simulink model "fft_biplex_real_4x_delay_bram_test"  (Simulink 7.4)
settings: Solver=VariableStepDiscrete  StartTime=0.0  StopTime=256  RelTol=1e-3
libraries: xbsIndex_r4 x596, casper_library_misc x36, casper_library_delays x8, casper_library_ffts_twiddle x1, simulink x1
(part 2 of 6)

== system fft_biplex_real_4x_delay_bram_test/fft_biplex_real_4x/bi_real_unscr_4x/hilbert0 ==
  a : Inport  OutDataType=sfix(16)  OutScaling=2^0
  b : Inport  Port=2  OutDataType=sfix(16)  OutScaling=2^0
  AddSub : xbsIndex_r4/AddSub  mode=Addition  use_carryin=off  use_carryout=off  en=off  latency=add_latency  precision=Full  arith_type=Unsigned  n_bits=8  bin_pt=2  quantization=Truncate  overflow=Wrap  dbl_ovrd=off  use_behavioral_HDL=on  hw_selection=Fabric  pipelined=off  use_rpm=on  block_type=addsub
      settings: xl_area=[0, 0, 0, 0, 0, 0, 0]  block_version=9.1.01
  AddSub1 : xbsIndex_r4/AddSub  mode=Subtraction  use_carryin=off  use_carryout=off  en=off  latency=add_latency  precision=Full  arith_type=Unsigned  n_bits=8  bin_pt=2  quantization=Truncate  overflow=Wrap  dbl_ovrd=off  use_behavioral_HDL=on  hw_selection=Fabric  pipelined=off  use_rpm=on  block_type=addsub
      settings: xl_area=[0, 0, 0, 0, 0, 0, 0]  block_version=9.1.01
  AddSub2 : xbsIndex_r4/AddSub  mode=Subtraction  use_carryin=off  use_carryout=off  en=off  latency=add_latency  precision=Full  arith_type=Unsigned  n_bits=8  bin_pt=2  quantization=Truncate  overflow=Wrap  dbl_ovrd=off  use_behavioral_HDL=on  hw_selection=Fabric  pipelined=off  use_rpm=on  block_type=addsub
      settings: xl_area=[0, 0, 0, 0, 0, 0, 0]  block_version=9.1.01
  AddSub3 : xbsIndex_r4/AddSub  mode=Addition  use_carryin=off  use_carryout=off  en=off  latency=add_latency  precision=Full  arith_type=Unsigned  n_bits=8  bin_pt=2  quantization=Truncate  overflow=Wrap  dbl_ovrd=off  use_behavioral_HDL=on  hw_selection=Fabric  pipelined=off  use_rpm=on  block_type=addsub
      settings: xl_area=[0, 0, 0, 0, 0, 0, 0]  block_version=9.1.01
  Convert{,1..3} (4 alike) : xbsIndex_r4/Convert  arith_type="Signed  (2's comp)"  n_bits=BitWidth  bin_pt=BitWidth - 1  quantization="Round  (unbiased: Even Values)"  overflow=Wrap  latency=conv_latency  dbl_ovrd=off  pipeline=off  block_type=convert
      settings: xl_area=[0, 0, 0, 0, 0, 0, 0]
  Scale{,1..3} (4 alike) : xbsIndex_r4/Scale  scale_factor=-1  dbl_ovrd=off  block_type=scale
  c_to_ri : Subsystem  AncestorBlock=casper_library_misc/c_to_ri  mask(c_to_ri){n_bits=BitWidth, bin_pt=BitWidth-1}
      mask prompts: n_bits "Bit Width"; bin_pt "Binary Point"
      mask help:
      | Outputs real and imaginary components of a complex input.
      | Useful for simplifying interconnects.
      | See also: Real-Imag to Complex (ri_to_c)
      mask init:
      | annotation=sprintf('%d_%d r/i',n_bits,bin_pt);
      | set_param(gcb,'AttributesFormatString',annotation);
      settings: AttributesFormatString=18_17 r/i
      mask Help: eval('xlWeb(''http://casper.berkeley.edu/wiki/C_to_ri'')')
  c_to_ri1 : Subsystem  AncestorBlock=casper_library_misc/c_to_ri  mask(c_to_ri){n_bits=BitWidth, bin_pt=BitWidth-1}
      mask prompts: n_bits "Bit Width"; bin_pt "Binary Point"
      mask help:
      | Outputs real and imaginary components of a complex input.
      | Useful for simplifying interconnects.
      | See also: Real-Imag to Complex (ri_to_c)
      mask init:
      | annotation=sprintf('%d_%d r/i',n_bits,bin_pt);
      | set_param(gcb,'AttributesFormatString',annotation);
      settings: AttributesFormatString=18_17 r/i
      mask Help: eval('xlWeb(''http://casper.berkeley.edu/wiki/C_to_ri'')')
  ri_to_c : Subsystem  AncestorBlock=casper_library_misc/ri_to_c
      mask Type: ri_to_c
      mask Description:
      | Concatenates real and imaginary inputs into a complex output.
      | Useful for simplifying interconnects.
      | See also: Complex to Real-Imag (c_to_ri)
      mask Help: eval('xlWeb(''http://casper.berkeley.edu/wiki/Ri_to_c'')')
  ri_to_c1 : Subsystem  AncestorBlock=casper_library_misc/ri_to_c
      mask Type: ri_to_c
      mask Description:
      | Concatenates real and imaginary inputs into a complex output.
      | Useful for simplifying interconnects.
      | See also: Complex to Real-Imag (c_to_ri)
      mask Help: eval('xlWeb(''http://casper.berkeley.edu/wiki/Ri_to_c'')')
  even : Outport  OutDataType=sfix(16)  OutScaling=2^0
  odd : Outport  Port=2  OutDataType=sfix(16)  OutScaling=2^0
  wires:
  Convert3/1 -> ri_to_c1/1(re)
  Convert1/1 -> ri_to_c1/2(im)
  AddSub/1 -> Scale/1
  AddSub1/1 -> Scale1/1
  AddSub2/1 -> Scale2/1
  AddSub3/1 -> Scale3/1
  c_to_ri/1(re) -> AddSub1/2, AddSub/1
  c_to_ri/2(im) -> AddSub2/1, AddSub3/1
  c_to_ri1/1(re) -> AddSub1/1, AddSub/2
  c_to_ri1/2(im) -> AddSub2/2, AddSub3/2
  Convert/1 -> ri_to_c/1(re)
  Convert2/1 -> ri_to_c/2(im)
  a/1 -> c_to_ri/1(c)
  ri_to_c/1(c) -> even/1
  ri_to_c1/1(c) -> odd/1
  b/1 -> c_to_ri1/1(c)
  Scale/1 -> Convert/1
  Scale1/1 -> Convert1/1
  Scale2/1 -> Convert2/1
  Scale3/1 -> Convert3/1

== system fft_biplex_real_4x_delay_bram_test/fft_biplex_real_4x/bi_real_unscr_4x/hilbert1 ==
  a : Inport  OutDataType=sfix(16)  OutScaling=2^0
  b : Inport  Port=2  OutDataType=sfix(16)  OutScaling=2^0
  AddSub : xbsIndex_r4/AddSub  mode=Addition  use_carryin=off  use_carryout=off  en=off  latency=add_latency  precision=Full  arith_type=Unsigned  n_bits=8  bin_pt=2  quantization=Truncate  overflow=Wrap  dbl_ovrd=off  use_behavioral_HDL=on  hw_selection=Fabric  pipelined=off  use_rpm=on  block_type=addsub
      settings: xl_area=[0, 0, 0, 0, 0, 0, 0]  block_version=9.1.01
  AddSub1 : xbsIndex_r4/AddSub  mode=Subtraction  use_carryin=off  use_carryout=off  en=off  latency=add_latency  precision=Full  arith_type=Unsigned  n_bits=8  bin_pt=2  quantization=Truncate  overflow=Wrap  dbl_ovrd=off  use_behavioral_HDL=on  hw_selection=Fabric  pipelined=off  use_rpm=on  block_type=addsub
      settings: xl_area=[0, 0, 0, 0, 0, 0, 0]  block_version=9.1.01
  AddSub2 : xbsIndex_r4/AddSub  mode=Subtraction  use_carryin=off  use_carryout=off  en=off  latency=add_latency  precision=Full  arith_type=Unsigned  n_bits=8  bin_pt=2  quantization=Truncate  overflow=Wrap  dbl_ovrd=off  use_behavioral_HDL=on  hw_selection=Fabric  pipelined=off  use_rpm=on  block_type=addsub
      settings: xl_area=[0, 0, 0, 0, 0, 0, 0]  block_version=9.1.01
  AddSub3 : xbsIndex_r4/AddSub  mode=Addition  use_carryin=off  use_carryout=off  en=off  latency=add_latency  precision=Full  arith_type=Unsigned  n_bits=8  bin_pt=2  quantization=Truncate  overflow=Wrap  dbl_ovrd=off  use_behavioral_HDL=on  hw_selection=Fabric  pipelined=off  use_rpm=on  block_type=addsub
      settings: xl_area=[0, 0, 0, 0, 0, 0, 0]  block_version=9.1.01
  Convert{,1..3} (4 alike) : xbsIndex_r4/Convert  arith_type="Signed  (2's comp)"  n_bits=BitWidth  bin_pt=BitWidth - 1  quantization="Round  (unbiased: Even Values)"  overflow=Wrap  latency=conv_latency  dbl_ovrd=off  pipeline=off  block_type=convert
      settings: xl_area=[0, 0, 0, 0, 0, 0, 0]
  Scale{,1..3} (4 alike) : xbsIndex_r4/Scale  scale_factor=-1  dbl_ovrd=off  block_type=scale
  c_to_ri : Subsystem  AncestorBlock=casper_library_misc/c_to_ri  mask(c_to_ri){n_bits=BitWidth, bin_pt=BitWidth-1}
      mask prompts: n_bits "Bit Width"; bin_pt "Binary Point"
      mask help:
      | Outputs real and imaginary components of a complex input.
      | Useful for simplifying interconnects.
      | See also: Real-Imag to Complex (ri_to_c)
      mask init:
      | annotation=sprintf('%d_%d r/i',n_bits,bin_pt);
      | set_param(gcb,'AttributesFormatString',annotation);
      settings: AttributesFormatString=18_17 r/i
      mask Help: eval('xlWeb(''http://casper.berkeley.edu/wiki/C_to_ri'')')
  c_to_ri1 : Subsystem  AncestorBlock=casper_library_misc/c_to_ri  mask(c_to_ri){n_bits=BitWidth, bin_pt=BitWidth-1}
      mask prompts: n_bits "Bit Width"; bin_pt "Binary Point"
      mask help:
      | Outputs real and imaginary components of a complex input.
      | Useful for simplifying interconnects.
      | See also: Real-Imag to Complex (ri_to_c)
      mask init:
      | annotation=sprintf('%d_%d r/i',n_bits,bin_pt);
      | set_param(gcb,'AttributesFormatString',annotation);
      settings: AttributesFormatString=18_17 r/i
      mask Help: eval('xlWeb(''http://casper.berkeley.edu/wiki/C_to_ri'')')
  ri_to_c : Subsystem  AncestorBlock=casper_library_misc/ri_to_c
      mask Type: ri_to_c
      mask Description:
      | Concatenates real and imaginary inputs into a complex output.
      | Useful for simplifying interconnects.
      | See also: Complex to Real-Imag (c_to_ri)
      mask Help: eval('xlWeb(''http://casper.berkeley.edu/wiki/Ri_to_c'')')
  ri_to_c1 : Subsystem  AncestorBlock=casper_library_misc/ri_to_c
      mask Type: ri_to_c
      mask Description:
      | Concatenates real and imaginary inputs into a complex output.
      | Useful for simplifying interconnects.
      | See also: Complex to Real-Imag (c_to_ri)
      mask Help: eval('xlWeb(''http://casper.berkeley.edu/wiki/Ri_to_c'')')
  even : Outport  OutDataType=sfix(16)  OutScaling=2^0
  odd : Outport  Port=2  OutDataType=sfix(16)  OutScaling=2^0
  wires:
  Convert3/1 -> ri_to_c1/1(re)
  Convert1/1 -> ri_to_c1/2(im)
  AddSub/1 -> Scale/1
  AddSub1/1 -> Scale1/1
  AddSub2/1 -> Scale2/1
  AddSub3/1 -> Scale3/1
  c_to_ri/1(re) -> AddSub1/2, AddSub/1
  c_to_ri/2(im) -> AddSub2/1, AddSub3/1
  c_to_ri1/1(re) -> AddSub1/1, AddSub/2
  c_to_ri1/2(im) -> AddSub2/2, AddSub3/2
  Convert/1 -> ri_to_c/1(re)
  Convert2/1 -> ri_to_c/2(im)
  a/1 -> c_to_ri/1(c)
  ri_to_c/1(c) -> even/1
  ri_to_c1/1(c) -> odd/1
  b/1 -> c_to_ri1/1(c)
  Scale/1 -> Convert/1
  Scale1/1 -> Convert1/1
  Scale2/1 -> Convert2/1
  Scale3/1 -> Convert3/1

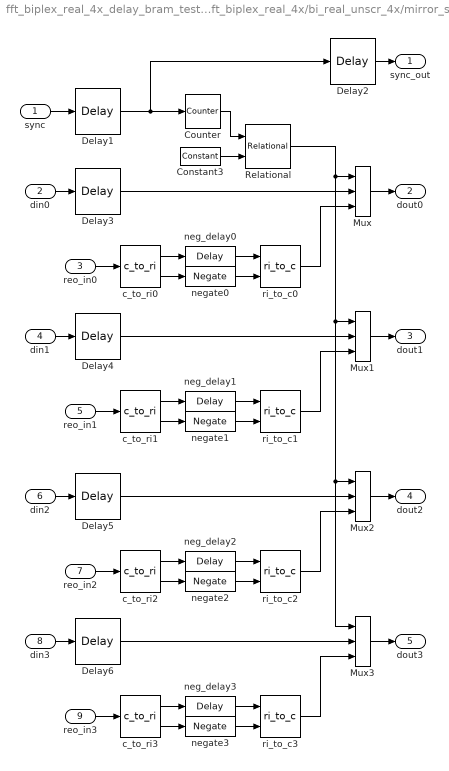
== system fft_biplex_real_4x_delay_bram_test/fft_biplex_real_4x/bi_real_unscr_4x/mirror_spectrum ==
  sync : Inport  OutDataType=sfix(16)  OutScaling=2^0
  din0 : Inport  Port=2  OutDataType=sfix(16)  OutScaling=2^0
  reo_in0 : Inport  Port=3  OutDataType=sfix(16)  OutScaling=2^0
  din1 : Inport  Port=4  OutDataType=sfix(16)  OutScaling=2^0
  reo_in1 : Inport  Port=5  OutDataType=sfix(16)  OutScaling=2^0
  din2 : Inport  Port=6  OutDataType=sfix(16)  OutScaling=2^0
  reo_in2 : Inport  Port=7  OutDataType=sfix(16)  OutScaling=2^0
  din3 : Inport  Port=8  OutDataType=sfix(16)  OutScaling=2^0
  reo_in3 : Inport  Port=9  OutDataType=sfix(16)  OutScaling=2^0
  Constant3 : xbsIndex_r4/Constant  arith_type=Unsigned  const=2^(FFTSize - 1)  n_bits=FFTSize  bin_pt=0  explicit_period=on  period=1  equ=P=C  opselect=C  inp2=PCIN>>17  opr=+  inp1=P  carry=CIN  dbl_ovrd=off  block_type=constant
      settings: block_version=9.1.01
  Counter : xbsIndex_r4/Counter  cnt_type=Free Running  cnt_to=Inf  operation=Up  start_count=0  cnt_by_val=1  arith_type=Unsigned  n_bits=FFTSize  bin_pt=0  load_pin=off  rst=on  en=off  explicit_period=off  period=1  dbl_ovrd=off  use_behavioral_HDL=off  implementation=Fabric  use_rpm=on  block_type=counter
      settings: xl_area=[0, 0, 0, 0, 0, 0, 0]  block_version=9.1.01
  Delay1 : xbsIndex_r4/Delay  en=off  latency=bram_latency - 2 + 1 + negate_latency  dbl_ovrd=off  reg_retiming=off  block_type=delay
      settings: xl_area=[0, 0, 0, 0, 0, 0, 0]  block_version=9.1.01
  Delay2 : xbsIndex_r4/Delay  en=off  latency=2  dbl_ovrd=off  reg_retiming=off  block_type=delay
      settings: xl_area=[0, 0, 0, 0, 0, 0, 0]  block_version=9.1.01
  Delay{3..6} (4 alike) : xbsIndex_r4/Delay  en=off  latency=bram_latency - 1 + 1 + negate_latency  dbl_ovrd=off  reg_retiming=off  block_type=delay
      settings: xl_area=[0, 0, 0, 0, 0, 0, 0]  block_version=9.1.01
  Mux{,1..3} (4 alike) : xbsIndex_r4/Mux  inputs=2  en=off  latency=1  precision=Full  arith_type="Signed  (2's comp)"  n_bits=8  bin_pt=2  quantization=Truncate  overflow=Wrap  dbl_ovrd=off  block_type=mux
      settings: xl_area=[0, 0, 0, 0, 0, 0, 0]  block_version=9.1.01
  Relational : xbsIndex_r4/Relational  mode=a>b  en=off  latency=1  dbl_ovrd=off  block_type=relational
      settings: xl_area=[0, 0, 0, 0, 0, 0, 0]  block_version=9.1.01
  c_to_ri{0..3} (4 alike) : casper_library_misc/c_to_ri  SystemSampleTime=-1  n_bits=input_bitwidth  bin_pt=input_bitwidth - 1
  neg_delay{0..3} (4 alike) : xbsIndex_r4/Delay  en=off  latency=negate_latency  dbl_ovrd=off  reg_retiming=off  block_type=delay
      settings: xl_area=[0, 0, 0, 0, 0, 0, 0]  block_version=9.1.01
  negate{0..3} (4 alike) : xbsIndex_r4/Negate  precision=User Defined  arith_type=Unsigned  n_bits=input_bit_width  bin_pt=input_bit_width - 1  quantization=Truncate  overflow=Wrap  en=off  latency=negate_latency  dbl_ovrd=off  block_type=negate
      settings: xl_area=[0, 0, 0, 0, 0, 0, 0]  block_version=9.1.01
  ri_to_c{0..3} (4 alike) : casper_library_misc/ri_to_c  SystemSampleTime=-1
  sync_out : Outport  OutDataType=sfix(16)  OutScaling=2^0
  dout0 : Outport  Port=2  OutDataType=sfix(16)  OutScaling=2^0
  dout1 : Outport  Port=3  OutDataType=sfix(16)  OutScaling=2^0
  dout2 : Outport  Port=4  OutDataType=sfix(16)  OutScaling=2^0
  dout3 : Outport  Port=5  OutDataType=sfix(16)  OutScaling=2^0
  wires:
  negate0/1 -> ri_to_c0/2
  c_to_ri0/2 -> negate0/1
  ri_to_c0/1 -> Mux/3
  c_to_ri0/1 -> neg_delay0/1
  reo_in0/1 -> c_to_ri0/1
  Delay2/1 -> sync_out/1
  Mux/1 -> dout0/1
  Delay1/1 -> Delay2/1, Counter/1
  Delay3/1 -> Mux/2
  din0/1 -> Delay3/1
  Relational/1 -> Mux/1, Mux1/1, Mux3/1, Mux2/1
  Constant3/1 -> Relational/2
  Counter/1 -> Relational/1
  sync/1 -> Delay1/1
  negate1/1 -> ri_to_c1/2
  c_to_ri1/2 -> negate1/1
  ri_to_c1/1 -> Mux1/3
  c_to_ri1/1 -> neg_delay1/1
  reo_in1/1 -> c_to_ri1/1
  Mux1/1 -> dout1/1
  Delay4/1 -> Mux1/2
  din1/1 -> Delay4/1
  negate2/1 -> ri_to_c2/2
  c_to_ri2/2 -> negate2/1
  ri_to_c2/1 -> Mux2/3
  c_to_ri2/1 -> neg_delay2/1
  reo_in2/1 -> c_to_ri2/1
  Mux2/1 -> dout2/1
  Delay5/1 -> Mux2/2
  din2/1 -> Delay5/1
  negate3/1 -> ri_to_c3/2
  c_to_ri3/2 -> negate3/1
  ri_to_c3/1 -> Mux3/3
  c_to_ri3/1 -> neg_delay3/1
  reo_in3/1 -> c_to_ri3/1
  Mux3/1 -> dout3/1
  Delay6/1 -> Mux3/2
  din3/1 -> Delay6/1
  neg_delay0/1 -> ri_to_c0/1
  neg_delay1/1 -> ri_to_c1/1
  neg_delay2/1 -> ri_to_c2/1
  neg_delay3/1 -> ri_to_c3/1

== system fft_biplex_real_4x_delay_bram_test/fft_biplex_real_4x/bi_real_unscr_4x/reorder_even ==
  sync : Inport  OutDataType=sfix(16)  OutScaling=2^0
  en : Inport  Port=2  OutDataType=sfix(16)  OutScaling=2^0
  din0 : Inport  Port=3  OutDataType=sfix(16)  OutScaling=2^0
  Counter : xbsIndex_r4/Counter  cnt_type=Count Limited  cnt_to=31  operation=Up  start_count=0  cnt_by_val=1  arith_type=Unsigned  n_bits=5  bin_pt=0  load_pin=off  rst=on  en=on  explicit_period=on  period=1  dbl_ovrd=off  use_behavioral_HDL=off  implementation=Fabric  block_type=counter
      settings: block_version=11.4
  Mux : xbsIndex_r4/Mux  inputs=2  en=off  latency=1  precision=Full  arith_type=Unsigned  n_bits=16  bin_pt=14  quantization=Truncate  overflow=Wrap  dbl_ovrd=off  block_type=mux
      settings: block_version=11.4
  Slice1 : xbsIndex_r4/Slice  nbits=1  boolean_output=off  mode=Upper Bit Location + Width  bit1=0  base1=MSB of Input  bit0=0  base0=LSB of Input  dbl_ovrd=off  block_type=slice
  Slice2 : xbsIndex_r4/Slice  nbits=4  boolean_output=off  mode=Lower Bit Location + Width  bit1=0  base1=MSB of Input  bit0=0  base0=LSB of Input  dbl_ovrd=off  block_type=slice
  bram0 : xbsIndex_r4/Single Port RAM  depth=16  initVector=sin(pi*(0:15)/16)  distributed_mem=Block RAM  write_mode=Read Before Write  rst=off  init_reg=0  en=off  latency=1  dbl_ovrd=off  optimize=Area  use_rpm=on  block_type=spram
  delay_d0 : xbsIndex_r4/Delay  en=off  latency=0  dbl_ovrd=off  reg_retiming=off  block_type=delay
      settings: block_version=11.4
  delay_din0 : xbsIndex_r4/Delay  en=off  latency=1  dbl_ovrd=off  reg_retiming=off  block_type=delay
      settings: xl_area=[0, 0, 0, 0, 0, 0, 0]  block_version=9.1.01
  delay_map1 : xbsIndex_r4/Delay  en=off  latency=0*map_latency  dbl_ovrd=off  reg_retiming=off  block_type=delay
      settings: block_version=11.4
  delay_sel : xbsIndex_r4/Delay  en=off  latency=0  dbl_ovrd=off  reg_retiming=off  block_type=delay
      settings: block_version=11.4
  delay_valid : xbsIndex_r4/Delay  en=off  latency=2  dbl_ovrd=off  reg_retiming=off  block_type=delay
      settings: xl_area=[0, 0, 0, 0, 0, 0, 0]  block_version=9.1.01
  delay_we : xbsIndex_r4/Delay  en=off  latency=0  dbl_ovrd=off  reg_retiming=off  block_type=delay
      settings: xl_area=[0, 0, 0, 0, 0, 0, 0]  block_version=9.1.01
  map1 : xbsIndex_r4/ROM  depth=16  initVector=map  distributed_mem=Distributed memory  rst=off  init_reg=0  en=off  latency=0  arith_type=Unsigned  n_bits=4  bin_pt=0  dbl_ovrd=off  optimize=Area  use_rpm=on  block_type=sprom
      settings: block_version=11.4
  post_sync_delay : xbsIndex_r4/Delay  en=off  latency=2  dbl_ovrd=off  reg_retiming=off  block_type=delay
      settings: xl_area=[0, 0, 0, 0, 0, 0, 0]  block_version=9.1.01
  pre_sync_delay : xbsIndex_r4/Delay  en=off  latency=0  dbl_ovrd=off  reg_retiming=off  block_type=delay
      settings: xl_area=[0, 0, 0, 0, 0, 0, 0]  block_version=9.1.01
  sync_delay_en : casper_library_delays/sync_delay_en  SystemSampleTime=-1  DelayLen=16
  sync_out : Outport  OutDataType=sfix(16)  OutScaling=2^0
  valid : Outport  Port=2  OutDataType=sfix(16)  OutScaling=2^0
  dout0 : Outport  Port=3  OutDataType=sfix(16)  OutScaling=2^0
  wires:
  sync/1 -> Counter/1, pre_sync_delay/1
  en/1 -> Counter/2, sync_delay_en/2, delay_we/1
  Counter/1 -> Slice1/1, Slice2/1
  Slice1/1 -> delay_sel/1
  delay_sel/1 -> Mux/1
  Slice2/1 -> delay_d0/1, map1/1
  delay_d0/1 -> Mux/2
  pre_sync_delay/1 -> sync_delay_en/1
  sync_delay_en/1 -> post_sync_delay/1
  post_sync_delay/1 -> sync_out/1
  delay_we/1 -> delay_valid/1, bram0/3
  delay_valid/1 -> valid/1
  Mux/1 -> bram0/1
  din0/1 -> delay_din0/1
  delay_din0/1 -> bram0/2
  bram0/1 -> dout0/1
  map1/1 -> delay_map1/1
  delay_map1/1 -> Mux/3

== system fft_biplex_real_4x_delay_bram_test/fft_biplex_real_4x/bi_real_unscr_4x/reorder_odd ==
  sync : Inport  OutDataType=sfix(16)  OutScaling=2^0
  en : Inport  Port=2  OutDataType=sfix(16)  OutScaling=2^0
  din0 : Inport  Port=3  OutDataType=sfix(16)  OutScaling=2^0
  Counter : xbsIndex_r4/Counter  cnt_type=Count Limited  cnt_to=31  operation=Up  start_count=0  cnt_by_val=1  arith_type=Unsigned  n_bits=5  bin_pt=0  load_pin=off  rst=on  en=on  explicit_period=on  period=1  dbl_ovrd=off  use_behavioral_HDL=off  implementation=Fabric  block_type=counter
      settings: block_version=11.4
  Mux : xbsIndex_r4/Mux  inputs=2  en=off  latency=1  precision=Full  arith_type=Unsigned  n_bits=16  bin_pt=14  quantization=Truncate  overflow=Wrap  dbl_ovrd=off  block_type=mux
      settings: block_version=11.4
  Slice1 : xbsIndex_r4/Slice  nbits=1  boolean_output=off  mode=Upper Bit Location + Width  bit1=0  base1=MSB of Input  bit0=0  base0=LSB of Input  dbl_ovrd=off  block_type=slice
  Slice2 : xbsIndex_r4/Slice  nbits=4  boolean_output=off  mode=Lower Bit Location + Width  bit1=0  base1=MSB of Input  bit0=0  base0=LSB of Input  dbl_ovrd=off  block_type=slice
  bram0 : xbsIndex_r4/Single Port RAM  depth=16  initVector=sin(pi*(0:15)/16)  distributed_mem=Block RAM  write_mode=Read Before Write  rst=off  init_reg=0  en=off  latency=1  dbl_ovrd=off  optimize=Area  use_rpm=on  block_type=spram
  delay_d0 : xbsIndex_r4/Delay  en=off  latency=0  dbl_ovrd=off  reg_retiming=off  block_type=delay
      settings: block_version=11.4
  delay_din0 : xbsIndex_r4/Delay  en=off  latency=1  dbl_ovrd=off  reg_retiming=off  block_type=delay
      settings: xl_area=[0, 0, 0, 0, 0, 0, 0]  block_version=9.1.01
  delay_map1 : xbsIndex_r4/Delay  en=off  latency=0*map_latency  dbl_ovrd=off  reg_retiming=off  block_type=delay
      settings: block_version=11.4
  delay_sel : xbsIndex_r4/Delay  en=off  latency=0  dbl_ovrd=off  reg_retiming=off  block_type=delay
      settings: block_version=11.4
  delay_valid : xbsIndex_r4/Delay  en=off  latency=2  dbl_ovrd=off  reg_retiming=off  block_type=delay
      settings: xl_area=[0, 0, 0, 0, 0, 0, 0]  block_version=9.1.01
  delay_we : xbsIndex_r4/Delay  en=off  latency=0  dbl_ovrd=off  reg_retiming=off  block_type=delay
      settings: xl_area=[0, 0, 0, 0, 0, 0, 0]  block_version=9.1.01
  map1 : xbsIndex_r4/ROM  depth=16  initVector=map  distributed_mem=Distributed memory  rst=off  init_reg=0  en=off  latency=0  arith_type=Unsigned  n_bits=4  bin_pt=0  dbl_ovrd=off  optimize=Area  use_rpm=on  block_type=sprom
      settings: block_version=11.4
  post_sync_delay : xbsIndex_r4/Delay  en=off  latency=2  dbl_ovrd=off  reg_retiming=off  block_type=delay
      settings: xl_area=[0, 0, 0, 0, 0, 0, 0]  block_version=9.1.01
  pre_sync_delay : xbsIndex_r4/Delay  en=off  latency=0  dbl_ovrd=off  reg_retiming=off  block_type=delay
      settings: xl_area=[0, 0, 0, 0, 0, 0, 0]  block_version=9.1.01
  sync_delay_en : casper_library_delays/sync_delay_en  SystemSampleTime=-1  DelayLen=16
  sync_out : Outport  OutDataType=sfix(16)  OutScaling=2^0
  valid : Outport  Port=2  OutDataType=sfix(16)  OutScaling=2^0
  dout0 : Outport  Port=3  OutDataType=sfix(16)  OutScaling=2^0
  wires:
  sync/1 -> Counter/1, pre_sync_delay/1
  en/1 -> Counter/2, sync_delay_en/2, delay_we/1
  Counter/1 -> Slice1/1, Slice2/1
  Slice1/1 -> delay_sel/1
  delay_sel/1 -> Mux/1
  Slice2/1 -> delay_d0/1, map1/1
  delay_d0/1 -> Mux/2
  pre_sync_delay/1 -> sync_delay_en/1
  sync_delay_en/1 -> post_sync_delay/1
  post_sync_delay/1 -> sync_out/1
  delay_we/1 -> delay_valid/1, bram0/3
  delay_valid/1 -> valid/1
  Mux/1 -> bram0/1
  din0/1 -> delay_din0/1
  delay_din0/1 -> bram0/2
  bram0/1 -> dout0/1
  map1/1 -> delay_map1/1
  delay_map1/1 -> Mux/3

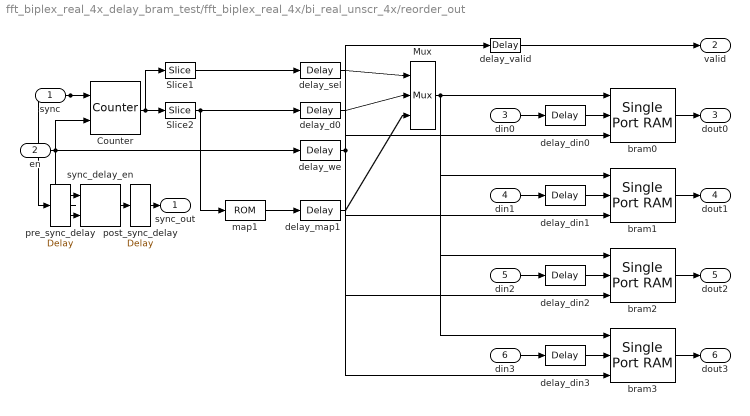
== system fft_biplex_real_4x_delay_bram_test/fft_biplex_real_4x/bi_real_unscr_4x/reorder_out ==
  sync : Inport  OutDataType=sfix(16)  OutScaling=2^0
  en : Inport  Port=2  OutDataType=sfix(16)  OutScaling=2^0
  din0 : Inport  Port=3  OutDataType=sfix(16)  OutScaling=2^0
  din1 : Inport  Port=4  OutDataType=sfix(16)  OutScaling=2^0
  din2 : Inport  Port=5
  din3 : Inport  Port=6
  Counter : xbsIndex_r4/Counter  cnt_type=Count Limited  cnt_to=31  operation=Up  start_count=0  cnt_by_val=1  arith_type=Unsigned  n_bits=5  bin_pt=0  load_pin=off  rst=on  en=on  explicit_period=on  period=1  dbl_ovrd=off  use_behavioral_HDL=off  implementation=Fabric  block_type=counter
      settings: block_version=11.4
  Mux : xbsIndex_r4/Mux  inputs=2  en=off  latency=1  precision=Full  arith_type=Unsigned  n_bits=16  bin_pt=14  quantization=Truncate  overflow=Wrap  dbl_ovrd=off  block_type=mux
      settings: block_version=11.4
  Slice1 : xbsIndex_r4/Slice  nbits=1  boolean_output=off  mode=Upper Bit Location + Width  bit1=0  base1=MSB of Input  bit0=0  base0=LSB of Input  dbl_ovrd=off  block_type=slice
  Slice2 : xbsIndex_r4/Slice  nbits=4  boolean_output=off  mode=Lower Bit Location + Width  bit1=0  base1=MSB of Input  bit0=0  base0=LSB of Input  dbl_ovrd=off  block_type=slice
  bram{0..3} (4 alike) : xbsIndex_r4/Single Port RAM  depth=16  initVector=sin(pi*(0:15)/16)  distributed_mem=Block RAM  write_mode=Read Before Write  rst=off  init_reg=0  en=off  latency=1  dbl_ovrd=off  optimize=Area  use_rpm=on  block_type=spram
  delay_d0 : xbsIndex_r4/Delay  en=off  latency=0  dbl_ovrd=off  reg_retiming=off  block_type=delay
      settings: block_version=11.4
  delay_din{0..3} (4 alike) : xbsIndex_r4/Delay  en=off  latency=1  dbl_ovrd=off  reg_retiming=off  block_type=delay
      delay_din0 settings: xl_area=[0, 0, 0, 0, 0, 0, 0]  block_version=9.1.01
      delay_din1 settings: xl_area=[0, 0, 0, 0, 0, 0, 0]  block_version=9.1.01
      delay_din2 settings: block_version=11.4
      delay_din3 settings: block_version=11.4
  delay_map1 : xbsIndex_r4/Delay  en=off  latency=0*map_latency  dbl_ovrd=off  reg_retiming=off  block_type=delay
      settings: block_version=11.4
  delay_sel : xbsIndex_r4/Delay  en=off  latency=0  dbl_ovrd=off  reg_retiming=off  block_type=delay
      settings: block_version=11.4
  delay_valid : xbsIndex_r4/Delay  en=off  latency=2  dbl_ovrd=off  reg_retiming=off  block_type=delay
      settings: xl_area=[0, 0, 0, 0, 0, 0, 0]  block_version=9.1.01
  delay_we : xbsIndex_r4/Delay  en=off  latency=0  dbl_ovrd=off  reg_retiming=off  block_type=delay
      settings: xl_area=[0, 0, 0, 0, 0, 0, 0]  block_version=9.1.01
  map1 : xbsIndex_r4/ROM  depth=16  initVector=map  distributed_mem=Distributed memory  rst=off  init_reg=0  en=off  latency=0  arith_type=Unsigned  n_bits=4  bin_pt=0  dbl_ovrd=off  optimize=Area  use_rpm=on  block_type=sprom
      settings: block_version=11.4
  post_sync_delay : xbsIndex_r4/Delay  en=off  latency=2  dbl_ovrd=off  reg_retiming=off  block_type=delay
      settings: xl_area=[0, 0, 0, 0, 0, 0, 0]  block_version=9.1.01
  pre_sync_delay : xbsIndex_r4/Delay  en=off  latency=0  dbl_ovrd=off  reg_retiming=off  block_type=delay
      settings: xl_area=[0, 0, 0, 0, 0, 0, 0]  block_version=9.1.01
  sync_delay_en : casper_library_delays/sync_delay_en  SystemSampleTime=-1  DelayLen=16
  sync_out : Outport  OutDataType=sfix(16)  OutScaling=2^0
  valid : Outport  Port=2  OutDataType=sfix(16)  OutScaling=2^0
  dout0 : Outport  Port=3  OutDataType=sfix(16)  OutScaling=2^0
  dout1 : Outport  Port=4  OutDataType=sfix(16)  OutScaling=2^0
  dout2 : Outport  Port=5
  dout3 : Outport  Port=6
  wires:
  sync/1 -> Counter/1, pre_sync_delay/1
  en/1 -> Counter/2, sync_delay_en/2, delay_we/1
  Counter/1 -> Slice1/1, Slice2/1
  Slice1/1 -> delay_sel/1
  delay_sel/1 -> Mux/1
  Slice2/1 -> delay_d0/1, map1/1
  delay_d0/1 -> Mux/2
  pre_sync_delay/1 -> sync_delay_en/1
  sync_delay_en/1 -> post_sync_delay/1
  post_sync_delay/1 -> sync_out/1
  delay_we/1 -> delay_valid/1, bram0/3, bram1/3, bram2/3, bram3/3
  delay_valid/1 -> valid/1
  Mux/1 -> bram0/1, bram1/1, bram2/1, bram3/1
  din0/1 -> delay_din0/1
  delay_din0/1 -> bram0/2
  bram0/1 -> dout0/1
  din1/1 -> delay_din1/1
  delay_din1/1 -> bram1/2
  bram1/1 -> dout1/1
  din2/1 -> delay_din2/1
  delay_din2/1 -> bram2/2
  bram2/1 -> dout2/1
  din3/1 -> delay_din3/1
  delay_din3/1 -> bram3/2
  bram3/1 -> dout3/1
  map1/1 -> delay_map1/1
  delay_map1/1 -> Mux/3

== system fft_biplex_real_4x_delay_bram_test/fft_biplex_real_4x/bi_real_unscr_4x/sync_delay_srl ==
  in : Inport  OutDataType=sfix(16)  OutScaling=2^0
  delay_ff : xbsIndex_r4/Delay  en=off  latency=ff_delay  dbl_ovrd=off  reg_retiming=off  block_type=delay
      settings: xl_area=[0, 0, 0, 0, 0, 0, 0]  block_version=9.1.01
  delay_srl : xbsIndex_r4/Delay  en=off  latency=srl_delay  dbl_ovrd=off  reg_retiming=off  block_type=delay
      settings: xl_area=[0, 0, 0, 0, 0, 0, 0]  block_version=9.1.01
  out : Outport  OutDataType=sfix(16)  OutScaling=2^0
  wires:
  delay_ff/1 -> delay_srl/1
  in/1 -> delay_ff/1
  delay_srl/1 -> out/1

== system fft_biplex_real_4x_delay_bram_test/fft_biplex_real_4x/biplex_core/fft_stage_1 ==
  in1 : Inport  OutDataType=sfix(16)  OutScaling=2^0
  in2 : Inport  Port=2  OutDataType=sfix(16)  OutScaling=2^0
  of_in : Inport  Port=3  OutDataType=sfix(16)  OutScaling=2^0
  sync : Inport  Port=4  OutDataType=sfix(16)  OutScaling=2^0
  shift : Inport  Port=5  OutDataType=sfix(16)  OutScaling=2^0
  Counter : xbsIndex_r4/Counter  cnt_type=Free Running  cnt_to=Inf  operation=Up  start_count=0  cnt_by_val=1  arith_type=Unsigned  n_bits=FFTSize-FFTStage+1  bin_pt=0  load_pin=off  rst=on  en=off  explicit_period=off  period=1  dbl_ovrd=off  use_behavioral_HDL=off  implementation=Fabric  use_rpm=off  block_type=counter
      settings: xl_area=[0, 0, 0, 0, 0, 0, 0]  block_version=9.1.01
  Delay : xbsIndex_r4/Delay  en=off  latency=1  dbl_ovrd=off  reg_retiming=off  block_type=delay
      settings: xl_area=[0, 0, 0, 0, 0, 0, 0]  block_version=9.1.01
  Logical1 : xbsIndex_r4/Logical  logical_function=OR  inputs=2  en=off  latency=1  precision=Full  arith_type=Unsigned  n_bits=8  bin_pt=2  align_bp=on  dbl_ovrd=off  block_type=logical
      settings: xl_area=[0, 0, 0, 0, 0, 0, 0]  block_version=9.1.01
  Mux : xbsIndex_r4/Mux  inputs=2  en=off  latency=1  precision=Full  arith_type="Signed  (2's comp)"  n_bits=8  bin_pt=2  quantization=Truncate  overflow=Wrap  dbl_ovrd=off  block_type=mux
      settings: xl_area=[0, 0, 0, 0, 0, 0, 0]  block_version=9.1.01
  Mux1 : xbsIndex_r4/Mux  inputs=2  en=off  latency=1  precision=Full  arith_type="Signed  (2's comp)"  n_bits=8  bin_pt=2  quantization=Truncate  overflow=Wrap  dbl_ovrd=off  block_type=mux
      settings: xl_area=[0, 0, 0, 0, 0, 0, 0]  block_version=9.1.01
  Slice : xbsIndex_r4/Slice  nbits=1  boolean_output=on  mode=Lower Bit Location + Width  bit1=-(FFTStage - 1)  base1=MSB of Input  bit0=FFTStage - 1  base0=LSB of Input  dbl_ovrd=off  block_type=slice
      settings: infoedit="Extracts a given range of bits from each input sample and presents it at the output.  The output type is ordinarily unsigned with binary point at zero, but can be Boolean when the slice is one bit wide.<P><P>Hardware notes: In hardware this block costs nothing."  block_version=9.1.01
  Slice1 : xbsIndex_r4/Slice  nbits=1  boolean_output=off  mode=Upper Bit Location + Width  bit1=0  base1=MSB of Input  bit0=0  base0=LSB of Input  dbl_ovrd=off  block_type=slice
      settings: infoedit="Extracts a given range of bits from each input sample and presents it at the output.  The output type is ordinarily unsigned with binary point at zero, but can be Boolean when the slice is one bit wide.<P><P>Hardware notes: In hardware this block costs nothing."  block_version=9.1.01
  butterfly_direct : Subsystem  AncestorBlock=casper_library_ffts/butterfly_direct  mask(butterfly_direct){biplex=on, FFTSize=5, Coeffs=0, StepPeriod=4, coeff_bit_width=16, input_bit_width=16, downshift=off, add_latency=1, mult_latency=3, bram_latency=1, conv_latency=2, quantization=Truncate, overflow=Saturate, arch=Virtex2Pro, opt_target=multipliers, coeffs_bram=off, use_hdl=on, use_embedded=off, hardcode_shifts=off, dsp48_adders=off}
      mask prompts: biplex "Used in biplex FFT"; FFTSize "Size of FFT: (2^? pts)"; Coeffs "Coefficients: (0 to 2^(FFTSize-1)-1)"; StepPeriod "Coefficient Step Period: (2^?)"; coeff_bit_width "Coefficient Bit Width"; input_bit_width "Input/Output Bit Width:"; add_latency "Add Latency"; mult_latency "Mult Latency"; bram_latency "BRAM Latency"; conv_latency "Convert latency"; quantization "Quantization Behavior"; overflow "Overflow Behavior"; arch "Architecture"; opt_target "Use less"; coeffs_bram "Store coefficients in BRAM"; use_hdl "Use behavioural HDL for multipliers"; use_embedded "Use embedded multipliers"; hardcode_shifts "Hardcode shift schedule"; dsp48_adders "Use DSP48s for adders"
      mask help: FFT internal block.
      mask init:
      | butterfly_direct_init(gcb, ...
      |     'biplex', biplex, ...
      |     'FFTSize', FFTSize, ...
      |     'Coeffs', Coeffs, ...
      |     'StepPeriod', StepPeriod, ...
      |     'coeff_bit_width', coeff_bit_width, ...
      |     'input_bit_width', input_bit_width, ...
      |     'hardcode_shifts', hardcode_shifts, ...
      |     'downshift', downshift, ...
      |     'add_latency', add_latency, ...
      |     'mult_latency', mult_latency, ...
      |     'bram_latency', bram_latency, ...
      |     'conv_latency', conv_latency, ...
      |     'quantization', quantization, ...
      |     'overflow', overflow, ...
      |     'arch', arch, ...
      |     'opt_target', opt_target, ...
      |     'coeffs_bram', coeffs_bram, ...    
      |     'use_hdl', use_hdl, ...
      |     'use_embedded', use_embedded, ...
      |     'dsp48_adders', dsp48_adders);
      settings: AttributesFormatString=|
      | twiddle_pass_through
      | coeffs in slices
      mask StyleString: checkbox,edit,edit,edit,edit,edit,checkbox,edit,edit,edit,edit,popup(Truncate|Round  (unbiased: +/- Inf)|Round  (unbiased: Even Values)),popup(Wrap|Saturate|Error),popup(Virtex2Pro|Virtex5),popup(logic|multipliers),checkbox,checkbox,checkbox,checkbox,checkbox
      mask CallbackString:
      | ||Coeffs = get_param(gcb, 'Coeffs');
      | if (length(eval(Coeffs)) == 1),
      |     set_param_state(gcb, 'StepPeriod', 'off');
      |     set_param_state(gcb, 'coeffs_bram', 'off');
      |     set_param_state(gcb, 'coeff_bit_width', 'off');
      | else
      |     set_param_state(gcb, 'StepPeriod', 'on');
      |     set_param_state(gcb, 'coeffs_bram', 'on');
      |     set_param_state(gcb, 'coeff_bit_width', 'on');
      | end|||||||||||fft_callback_arch(gcb);|||% make mutually exclusive with use_embedded.
      | 
      | use_hdl = get_param(gcb, 'use_hdl');
      | if strcmp(use_hdl, 'on'),
      |     set_param_state(gcb, 'use_embedded', 'off');
      | else
      |     set_param_state(gcb, 'use_embedded', 'on');
      | end|% make mutually exclusive with use_hdl.
      | 
      | use_hdl = get_param(gcb, 'use_embedded');
      | if strcmp(use_hdl, 'on'),
      |     set_param_state(gcb, 'use_hdl', 'off');
      | else
      |     set_param_state(gcb, 'use_hdl', 'on');
      | end|hardcode_shifts = get_param(gcb, 'hardcode_shifts');
      | set_param_state(gcb, 'downshift', hardcode_shifts);|fft_callback_dsp48_adders(gcb);
      mask TabNameString: Basic,Basic,Basic,Basic,Basic,Basic,Basic,Latency,Latency,Latency,Latency,Implementation,Implementation,Implementation,Implementation,Implementation,Implementation,Implementation,Implementation,Implementation
  delay_b : Subsystem  AncestorBlock=casper_library_delays/delay_slr  mask(delay_slr){DelayLen=2^(FFTSize-FFTStage)}
      mask prompts: DelayLen "Delay by:"
      mask help: A delay block that uses slices (SLR16s) for its storage.
      mask Help: eval('xlWeb(''http://casper.berkeley.edu/wiki/Delay_slr'')')
  delay_f : Subsystem  AncestorBlock=casper_library_delays/delay_slr  mask(delay_slr){DelayLen=2^(FFTSize-FFTStage)}
      mask prompts: DelayLen "Delay by:"
      mask help: A delay block that uses slices (SLR16s) for its storage.
      mask Help: eval('xlWeb(''http://casper.berkeley.edu/wiki/Delay_slr'')')
  sync_delay : casper_library_delays/sync_delay  SystemSampleTime=-1  DelayLen=2^(FFTSize - FFTStage)
  out1 : Outport  OutDataType=sfix(16)  OutScaling=2^0
  out2 : Outport  Port=2  OutDataType=sfix(16)  OutScaling=2^0
  of : Outport  Port=3  OutDataType=sfix(16)  OutScaling=2^0
  sync_out : Outport  Port=4  OutDataType=sfix(16)  OutScaling=2^0
  wires:
  shift/1 -> Slice/1
  of_in/1 -> Logical1/2
  Logical1/1 -> of/1
  Delay/1 -> sync_delay/1
  sync/1 -> Counter/1, Delay/1
  Counter/1 -> Slice1/1
  Mux/1 -> butterfly_direct/2(b)
  Mux1/1 -> delay_b/1(In1)
  delay_f/1(Out1) -> Mux1/3, Mux/2
  in1/1 -> Mux/3, Mux1/2
  Slice1/1 -> Mux/1, Mux1/1
  in2/1 -> delay_f/1(In1)
  delay_b/1(Out1) -> butterfly_direct/1(a)
  sync_delay/1 -> butterfly_direct/3(sync)
  Slice/1 -> butterfly_direct/4(shift)
  butterfly_direct/1(a+bw) -> out1/1
  butterfly_direct/2(a-bw) -> out2/1
  butterfly_direct/3(of) -> Logical1/1
  butterfly_direct/4(sync_out) -> sync_out/1

== system fft_biplex_real_4x_delay_bram_test/fft_biplex_real_4x/biplex_core/fft_stage_2 ==
  in1 : Inport  OutDataType=sfix(16)  OutScaling=2^0
  in2 : Inport  Port=2  OutDataType=sfix(16)  OutScaling=2^0
  of_in : Inport  Port=3  OutDataType=sfix(16)  OutScaling=2^0
  sync : Inport  Port=4  OutDataType=sfix(16)  OutScaling=2^0
  shift : Inport  Port=5  OutDataType=sfix(16)  OutScaling=2^0
  Counter : xbsIndex_r4/Counter  cnt_type=Free Running  cnt_to=Inf  operation=Up  start_count=0  cnt_by_val=1  arith_type=Unsigned  n_bits=FFTSize-FFTStage+1  bin_pt=0  load_pin=off  rst=on  en=off  explicit_period=off  period=1  dbl_ovrd=off  use_behavioral_HDL=off  implementation=Fabric  use_rpm=off  block_type=counter
      settings: xl_area=[0, 0, 0, 0, 0, 0, 0]  block_version=9.1.01
  Delay : xbsIndex_r4/Delay  en=off  latency=1  dbl_ovrd=off  reg_retiming=off  block_type=delay
      settings: xl_area=[0, 0, 0, 0, 0, 0, 0]  block_version=9.1.01
  Logical1 : xbsIndex_r4/Logical  logical_function=OR  inputs=2  en=off  latency=1  precision=Full  arith_type=Unsigned  n_bits=8  bin_pt=2  align_bp=on  dbl_ovrd=off  block_type=logical
      settings: xl_area=[0, 0, 0, 0, 0, 0, 0]  block_version=9.1.01
  Mux : xbsIndex_r4/Mux  inputs=2  en=off  latency=1  precision=Full  arith_type="Signed  (2's comp)"  n_bits=8  bin_pt=2  quantization=Truncate  overflow=Wrap  dbl_ovrd=off  block_type=mux
      settings: xl_area=[0, 0, 0, 0, 0, 0, 0]  block_version=9.1.01
  Mux1 : xbsIndex_r4/Mux  inputs=2  en=off  latency=1  precision=Full  arith_type="Signed  (2's comp)"  n_bits=8  bin_pt=2  quantization=Truncate  overflow=Wrap  dbl_ovrd=off  block_type=mux
      settings: xl_area=[0, 0, 0, 0, 0, 0, 0]  block_version=9.1.01
  Slice : xbsIndex_r4/Slice  nbits=1  boolean_output=on  mode=Lower Bit Location + Width  bit1=-(FFTStage - 1)  base1=MSB of Input  bit0=FFTStage - 1  base0=LSB of Input  dbl_ovrd=off  block_type=slice
      settings: infoedit="Extracts a given range of bits from each input sample and presents it at the output.  The output type is ordinarily unsigned with binary point at zero, but can be Boolean when the slice is one bit wide.<P><P>Hardware notes: In hardware this block costs nothing."  block_version=9.1.01
  Slice1 : xbsIndex_r4/Slice  nbits=1  boolean_output=off  mode=Upper Bit Location + Width  bit1=0  base1=MSB of Input  bit0=0  base0=LSB of Input  dbl_ovrd=off  block_type=slice
      settings: infoedit="Extracts a given range of bits from each input sample and presents it at the output.  The output type is ordinarily unsigned with binary point at zero, but can be Boolean when the slice is one bit wide.<P><P>Hardware notes: In hardware this block costs nothing."  block_version=9.1.01
  butterfly_direct : Subsystem  AncestorBlock=casper_library_ffts/butterfly_direct  mask(butterfly_direct){biplex=on, FFTSize=5, Coeffs=[0                                      1], StepPeriod=3, coeff_bit_width=16, input_bit_width=16, downshift=off, add_latency=1, mult_latency=3, bram_latency=1, conv_latency=2, quantization=Truncate, overflow=Saturate, arch=Virtex2Pro, opt_target=multipliers, coeffs_bram=off, use_hdl=off, use_embedded=on, hardcode_shifts=off, dsp48_adders=off}
      mask prompts: biplex "Used in biplex FFT"; FFTSize "Size of FFT: (2^? pts)"; Coeffs "Coefficients: (0 to 2^(FFTSize-1)-1)"; StepPeriod "Coefficient Step Period: (2^?)"; coeff_bit_width "Coefficient Bit Width"; input_bit_width "Input/Output Bit Width:"; add_latency "Add Latency"; mult_latency "Mult Latency"; bram_latency "BRAM Latency"; conv_latency "Convert latency"; quantization "Quantization Behavior"; overflow "Overflow Behavior"; arch "Architecture"; opt_target "Use less"; coeffs_bram "Store coefficients in BRAM"; use_hdl "Use behavioural HDL for multipliers"; use_embedded "Use embedded multipliers"; hardcode_shifts "Hardcode shift schedule"; dsp48_adders "Use DSP48s for adders"
      mask help: FFT internal block.
      mask init: same as fft_biplex_real_4x_delay_bram_test/fft_biplex_real_4x/biplex_core/fft_stage_1/butterfly_direct
      settings: AttributesFormatString=|
      | twiddle_stage_2
      | coeffs in slices
      mask StyleString: checkbox,edit,edit,edit,edit,edit,checkbox,edit,edit,edit,edit,popup(Truncate|Round  (unbiased: +/- Inf)|Round  (unbiased: Even Values)),popup(Wrap|Saturate|Error),popup(Virtex2Pro|Virtex5),popup(logic|multipliers),checkbox,checkbox,checkbox,checkbox,checkbox
      mask CallbackString:
      | ||Coeffs = get_param(gcb, 'Coeffs');
      | if (length(eval(Coeffs)) == 1),
      |     set_param_state(gcb, 'StepPeriod', 'off');
      |     set_param_state(gcb, 'coeffs_bram', 'off');
      |     set_param_state(gcb, 'coeff_bit_width', 'off');
      | else
      |     set_param_state(gcb, 'StepPeriod', 'on');
      |     set_param_state(gcb, 'coeffs_bram', 'on');
      |     set_param_state(gcb, 'coeff_bit_width', 'on');
      | end|||||||||||fft_callback_arch(gcb);|||% make mutually exclusive with use_embedded.
      | 
      | use_hdl = get_param(gcb, 'use_hdl');
      | if strcmp(use_hdl, 'on'),
      |     set_param_state(gcb, 'use_embedded', 'off');
      | else
      |     set_param_state(gcb, 'use_embedded', 'on');
      | end|% make mutually exclusive with use_hdl.
      | 
      | use_hdl = get_param(gcb, 'use_embedded');
      | if strcmp(use_hdl, 'on'),
      |     set_param_state(gcb, 'use_hdl', 'off');
      | else
      |     set_param_state(gcb, 'use_hdl', 'on');
      | end|hardcode_shifts = get_param(gcb, 'hardcode_shifts');
      | set_param_state(gcb, 'downshift', hardcode_shifts);|fft_callback_dsp48_adders(gcb);
      mask TabNameString: Basic,Basic,Basic,Basic,Basic,Basic,Basic,Latency,Latency,Latency,Latency,Implementation,Implementation,Implementation,Implementation,Implementation,Implementation,Implementation,Implementation,Implementation
  delay_b : Subsystem  AncestorBlock=casper_library_delays/delay_slr  mask(delay_slr){DelayLen=2^(FFTSize-FFTStage)}
      mask prompts: DelayLen "Delay by:"
      mask help: A delay block that uses slices (SLR16s) for its storage.
      mask Help: eval('xlWeb(''http://casper.berkeley.edu/wiki/Delay_slr'')')
  delay_f : Subsystem  AncestorBlock=casper_library_delays/delay_slr  mask(delay_slr){DelayLen=2^(FFTSize-FFTStage)}
      mask prompts: DelayLen "Delay by:"
      mask help: A delay block that uses slices (SLR16s) for its storage.
      mask Help: eval('xlWeb(''http://casper.berkeley.edu/wiki/Delay_slr'')')
  sync_delay : casper_library_delays/sync_delay  SystemSampleTime=-1  DelayLen=2^(FFTSize - FFTStage)
  out1 : Outport  OutDataType=sfix(16)  OutScaling=2^0
  out2 : Outport  Port=2  OutDataType=sfix(16)  OutScaling=2^0
  of : Outport  Port=3  OutDataType=sfix(16)  OutScaling=2^0
  sync_out : Outport  Port=4  OutDataType=sfix(16)  OutScaling=2^0
  wires:
  shift/1 -> Slice/1
  of_in/1 -> Logical1/2
  Logical1/1 -> of/1
  Delay/1 -> sync_delay/1
  sync/1 -> Counter/1, Delay/1
  Counter/1 -> Slice1/1
  Mux/1 -> butterfly_direct/2(b)
  Mux1/1 -> delay_b/1(In1)
  delay_f/1(Out1) -> Mux1/3, Mux/2
  in1/1 -> Mux/3, Mux1/2
  Slice1/1 -> Mux/1, Mux1/1
  in2/1 -> delay_f/1(In1)
  delay_b/1(Out1) -> butterfly_direct/1(a)
  sync_delay/1 -> butterfly_direct/3(sync)
  Slice/1 -> butterfly_direct/4(shift)
  butterfly_direct/1(a+bw) -> out1/1
  butterfly_direct/2(a-bw) -> out2/1
  butterfly_direct/3(of) -> Logical1/1
  butterfly_direct/4(sync_out) -> sync_out/1
